simulink model "ATOM_simple_planning_simulator"  (R2026a)
settings: Solver=ode4  StopTime=100  FixedStep=0.01
StopFcn:
  | % Put every new figure in the same MATLAB Figures window as a docked tab.
  | set(groot, 'defaultFigureWindowStyle', 'docked');
  | 
  | if exist('costmap_active', 'var') && ...
  |     exist('vehicle', 'var') && ...
  |     exist('parking_path', 'var') && ...
  |     ~isempty(parking_path)
  | 
  |      plotPlan(costmap_active, vehicle, parking_path);
  | 
  |  else
  | 
  |      warning('No valid parking path is available for plotting.');
  | 
  |  end
  | 
  |  PlotControllerReferences( ...
  |      out.controller_reference_log);
  | 
  |  PlotControllerTracking( ...
  |      out.controller_tracking_log);
  | 
model workspace (MAT data in the model file):
  vehicle : object (value not decoded)
symbols that are objects in the model workspace (value not decoded): vehicle
undefined symbols (not defined in the file): delta_f_LUT, gain4WS_LUT, k_ref_LUT, kappa_gain_BP, Ki, Kp, lateral, longitudinal, planning_validator, rr_gain_BP, rr_LUT, stanley, velocity_smoother
libraries: slpidlib x1
(part 2 of 8)

== system ATOM_simple_planning_simulator/Lateral run()/SetStanleyTrajectory ==
  ref_traj : Inport
  ego_pose : Inport  Port=2
  Constant1 : Constant  Value=stanley.traj_resample_dist
  Resample Trajectory : MATLAB Function  TreatAsAtomicUnit=on
  calcLongOffsetToSegment : MATLAB Function  TreatAsAtomicUnit=on
  default : Constant  Value=3
  default1 : Constant  Value=pi/2
  findFirstNearestSegmentIndexWithSoftConstraints : MATLAB Function  TreatAsAtomicUnit=on
  trajectory_out : Outport
  wires:
  Constant1/1 -> Resample Trajectory/2(resample_interval_dist)
  calcLongOffsetToSegment/1(ego_offset_to_segment) -> Resample Trajectory/4(ego_offset_to_segment)
  ego_pose/1 -> findFirstNearestSegmentIndexWithSoftConstraints/4(pose), calcLongOffsetToSegment/2(ego_pose)
  findFirstNearestSegmentIndexWithSoftConstraints/1(nearest_seg_idx) -> calcLongOffsetToSegment/1(seg_idx), Resample Trajectory/3(nearest_seg_idx)
  default/1 -> findFirstNearestSegmentIndexWithSoftConstraints/2(dist_threshold)
  default1/1 -> findFirstNearestSegmentIndexWithSoftConstraints/3(yaw_threshold)
  Resample Trajectory/1(trajectory_out) -> trajectory_out/1
  ref_traj/1 -> Resample Trajectory/1(trajectory_in), calcLongOffsetToSegment/3(trajectory), findFirstNearestSegmentIndexWithSoftConstraints/1(trajectory)

== system ATOM_simple_planning_simulator/Parking Scenario2/Costmap generation: complex parking situation ==
  From Workspace1 : FromWorkspace  VariableName=veh
  MATLAB Function : MATLAB Function  TreatAsAtomicUnit=on
  costmap : Outport
  start_pose : Outport  Port=2
  goal_pose : Outport  Port=3
  wires:
  MATLAB Function/1(costmap) -> costmap/1
  From Workspace1/1 -> MATLAB Function/1(veh)
  MATLAB Function/2(start_pose) -> start_pose/1
  MATLAB Function/3(goal_pose) -> goal_pose/1

== system ATOM_simple_planning_simulator/Parking Scenario2/Costmap generation: corridor occupancy grid ==
  From Workspace1 : FromWorkspace  VariableName=veh
  MATLAB Function : MATLAB Function  TreatAsAtomicUnit=on
  costmap : Outport
  start_pose : Outport  Port=2
  goal_pose : Outport  Port=3
  wires:
  MATLAB Function/1(costmap) -> costmap/1
  From Workspace1/1 -> MATLAB Function/1(veh)
  MATLAB Function/3(goal_pose) -> goal_pose/1
  MATLAB Function/2(start_pose) -> start_pose/1

== system ATOM_simple_planning_simulator/Parking Scenario2/Costmap generation: empty occupancy grid ==
  From Workspace1 : FromWorkspace  VariableName=veh
  MATLAB Function : MATLAB Function  TreatAsAtomicUnit=on
  costmap : Outport
  start_pose : Outport  Port=2
  goal_pose : Outport  Port=3
  wires:
  MATLAB Function/1(costmap) -> costmap/1
  From Workspace1/1 -> MATLAB Function/1(veh)
  MATLAB Function/2(start_pose) -> start_pose/1
  MATLAB Function/3(goal_pose) -> goal_pose/1

== system ATOM_simple_planning_simulator/Parking Scenario2/Costmap generation: obstacle ==
  From Workspace1 : FromWorkspace  VariableName=veh
  MATLAB Function : MATLAB Function  TreatAsAtomicUnit=on
  costmap : Outport
  start_pose : Outport  Port=2
  goal_pose : Outport  Port=3
  wires:
  MATLAB Function/1(costmap) -> costmap/1
  From Workspace1/1 -> MATLAB Function/1(veh)
  MATLAB Function/2(start_pose) -> start_pose/1
  MATLAB Function/3(goal_pose) -> goal_pose/1

== system ATOM_simple_planning_simulator/Parking Scenario2/Costmap generation: obstacle1 ==
  From Workspace1 : FromWorkspace  VariableName=veh
  MATLAB Function : MATLAB Function  TreatAsAtomicUnit=on
  costmap : Outport
  start_pose : Outport  Port=2
  goal_pose : Outport  Port=3
  wires:
  MATLAB Function/1(costmap) -> costmap/1
  From Workspace1/1 -> MATLAB Function/1(veh)
  MATLAB Function/2(start_pose) -> start_pose/1
  MATLAB Function/3(goal_pose) -> goal_pose/1

== system ATOM_simple_planning_simulator/Parking Scenario2/Costmap generation: obstacle2 ==
  From Workspace1 : FromWorkspace  VariableName=veh
  MATLAB Function : MATLAB Function  TreatAsAtomicUnit=on
  costmap : Outport
  start_pose : Outport  Port=2
  goal_pose : Outport  Port=3
  wires:
  MATLAB Function/1(costmap) -> costmap/1
  From Workspace1/1 -> MATLAB Function/1(veh)
  MATLAB Function/2(start_pose) -> start_pose/1
  MATLAB Function/3(goal_pose) -> goal_pose/1

== system ATOM_simple_planning_simulator/Parking Scenario2/Costmap generation: parking scenario beside a lane ==
  From Workspace1 : FromWorkspace  VariableName=veh
  MATLAB Function : MATLAB Function  TreatAsAtomicUnit=on
  costmap : Outport
  start_pose : Outport  Port=2
  goal_pose : Outport  Port=3
  wires:
  MATLAB Function/1(costmap) -> costmap/1
  From Workspace1/1 -> MATLAB Function/1(veh)
  MATLAB Function/2(start_pose) -> start_pose/1
  MATLAB Function/3(goal_pose) -> goal_pose/1

== system ATOM_simple_planning_simulator/Parking Scenario2/Costmap generation: perpendicular lot ==
  From Workspace1 : FromWorkspace  VariableName=veh
  Perpendicular Parking : MATLAB Function  TreatAsAtomicUnit=on
  costmap : Outport
  start_pose : Outport  Port=2
  goal_pose : Outport  Port=3
  wires:
  Perpendicular Parking/1(costmap) -> costmap/1
  From Workspace1/1 -> Perpendicular Parking/1(veh)
  Perpendicular Parking/2(start_pose) -> start_pose/1
  Perpendicular Parking/3(goal_pose) -> goal_pose/1

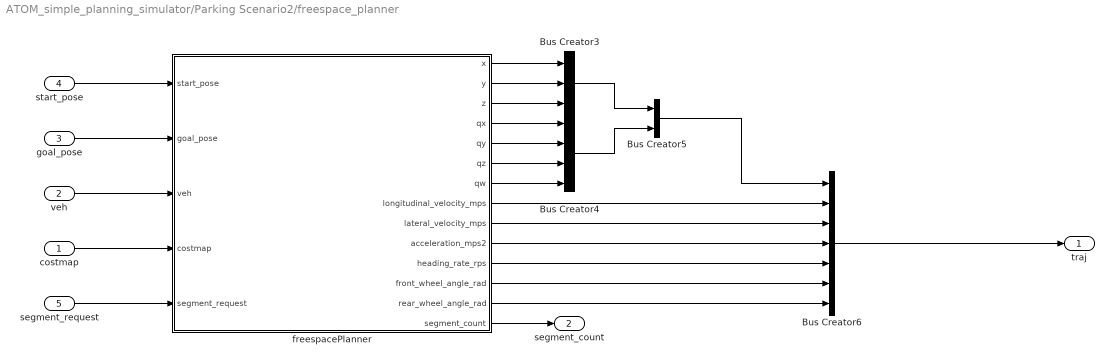
== system ATOM_simple_planning_simulator/Parking Scenario2/freespace_planner ==
  costmap : Inport
  veh : Inport  Port=2
  goal_pose : Inport  Port=3
  start_pose : Inport  Port=4
  segment_request : Inport  Port=5
  Bus Creator3 : BusCreator  Inputs=3  OutDataTypeStr=Bus: PointBusN
  Bus Creator4 : BusCreator  Inputs=4  OutDataTypeStr=Bus: QuaternionBusN
  Bus Creator5 : BusCreator  Inputs=2  OutDataTypeStr=Bus: PoseBusN
      settings: InheritFromInputs=off
  Bus Creator6 : BusCreator  Inputs=7  OutDataTypeStr=Bus: TrajectoryDataBus
      settings: InheritFromInputs=off
  freespacePlanner : MATLAB Function  TreatAsAtomicUnit=on
  traj : Outport
  segment_count : Outport  Port=2
  wires:
  Bus Creator6/1 -> traj/1
  Bus Creator3/1 -> Bus Creator5/1
  freespacePlanner/13(rear_wheel_angle_rad) -> Bus Creator6/7
  Bus Creator5/1 -> Bus Creator6/1
  freespacePlanner/8(longitudinal_velocity_mps) -> Bus Creator6/2
  freespacePlanner/3(z) -> Bus Creator3/3
  freespacePlanner/4(qx) -> Bus Creator4/1
  freespacePlanner/9(lateral_velocity_mps) -> Bus Creator6/3
  freespacePlanner/10(acceleration_mps2) -> Bus Creator6/4
  freespacePlanner/5(qy) -> Bus Creator4/2
  freespacePlanner/1(x) -> Bus Creator3/1
  freespacePlanner/2(y) -> Bus Creator3/2
  freespacePlanner/7(qw) -> Bus Creator4/4
  freespacePlanner/6(qz) -> Bus Creator4/3
  freespacePlanner/12(front_wheel_angle_rad) -> Bus Creator6/6
  Bus Creator4/1 -> Bus Creator5/2
  freespacePlanner/11(heading_rate_rps) -> Bus Creator6/5
  costmap/1 -> freespacePlanner/4(costmap)
  start_pose/1 -> freespacePlanner/1(start_pose)
  goal_pose/1 -> freespacePlanner/2(goal_pose)
  veh/1 -> freespacePlanner/3(veh)
  segment_request/1 -> freespacePlanner/5(segment_request)
  freespacePlanner/14(segment_count) -> segment_count/1

== system ATOM_simple_planning_simulator/Plot vehicle/SetStanleyTrajectory ==
  ref_traj : Inport
  ego_pose : Inport  Port=2
  Constant1 : Constant  Value=stanley.traj_resample_dist
  Resample Trajectory : MATLAB Function  TreatAsAtomicUnit=on
  calcLongOffsetToSegment : MATLAB Function  TreatAsAtomicUnit=on
  default : Constant  Value=3
  default1 : Constant  Value=pi/2
  findFirstNearestSegmentIndexWithSoftConstraints : MATLAB Function  TreatAsAtomicUnit=on
  trajectory_out : Outport
  wires:
  ref_traj/1 -> Resample Trajectory/1(trajectory_in), calcLongOffsetToSegment/3(trajectory), findFirstNearestSegmentIndexWithSoftConstraints/1(trajectory)
  Constant1/1 -> Resample Trajectory/2(resample_interval_dist)
  calcLongOffsetToSegment/1(ego_offset_to_segment) -> Resample Trajectory/4(ego_offset_to_segment)
  ego_pose/1 -> findFirstNearestSegmentIndexWithSoftConstraints/4(pose), calcLongOffsetToSegment/2(ego_pose)
  findFirstNearestSegmentIndexWithSoftConstraints/1(nearest_seg_idx) -> calcLongOffsetToSegment/1(seg_idx), Resample Trajectory/3(nearest_seg_idx)
  default/1 -> findFirstNearestSegmentIndexWithSoftConstraints/2(dist_threshold)
  default1/1 -> findFirstNearestSegmentIndexWithSoftConstraints/3(yaw_threshold)
  Resample Trajectory/1(trajectory_out) -> trajectory_out/1

== system ATOM_simple_planning_simulator/Plot vehicle3/SetStanleyTrajectory ==
  ref_traj : Inport
  ego_pose : Inport  Port=2
  Constant1 : Constant  Value=stanley.traj_resample_dist
  Resample Trajectory : MATLAB Function  TreatAsAtomicUnit=on
  calcLongOffsetToSegment : MATLAB Function  TreatAsAtomicUnit=on
  default : Constant  Value=3
  default1 : Constant  Value=pi/2
  findFirstNearestSegmentIndexWithSoftConstraints : MATLAB Function  TreatAsAtomicUnit=on
  trajectory_out : Outport
  wires:
  ref_traj/1 -> Resample Trajectory/1(trajectory_in), calcLongOffsetToSegment/3(trajectory), findFirstNearestSegmentIndexWithSoftConstraints/1(trajectory)
  Constant1/1 -> Resample Trajectory/2(resample_interval_dist)
  calcLongOffsetToSegment/1(ego_offset_to_segment) -> Resample Trajectory/4(ego_offset_to_segment)
  ego_pose/1 -> findFirstNearestSegmentIndexWithSoftConstraints/4(pose), calcLongOffsetToSegment/2(ego_pose)
  findFirstNearestSegmentIndexWithSoftConstraints/1(nearest_seg_idx) -> calcLongOffsetToSegment/1(seg_idx), Resample Trajectory/3(nearest_seg_idx)
  default/1 -> findFirstNearestSegmentIndexWithSoftConstraints/2(dist_threshold)
  default1/1 -> findFirstNearestSegmentIndexWithSoftConstraints/3(yaw_threshold)
  Resample Trajectory/1(trajectory_out) -> trajectory_out/1

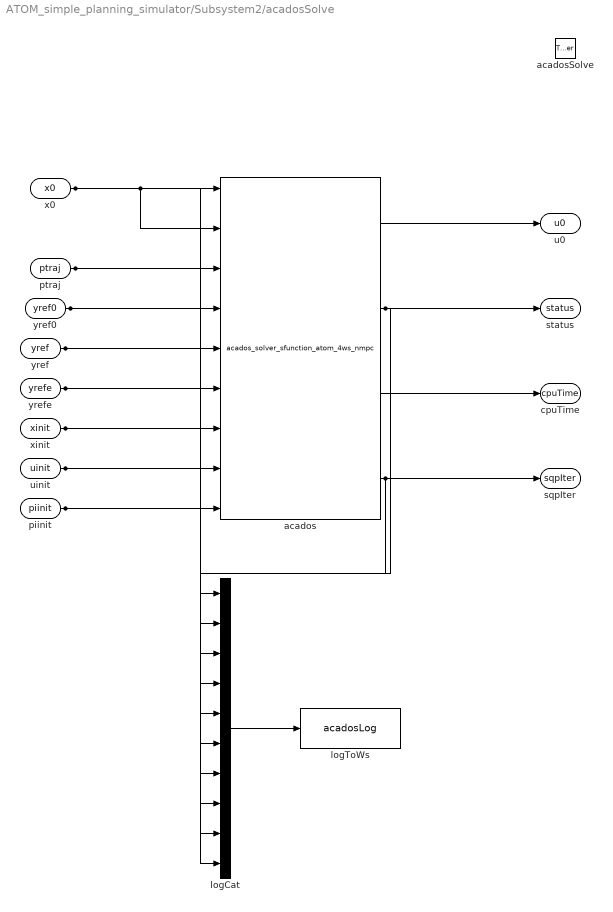
== system ATOM_simple_planning_simulator/Subsystem2/acadosSolve ==
  acadosSolve : TriggerPort  TriggerType=function-call  IsSimulinkFunction=on  FunctionName=acadosSolve  FunctionVisibility=scoped  VariantControl=(inherit)
  acados : S-Function  FunctionName=acados_solver_sfunction_atom_4ws_nmpc  SFunctionDeploymentMode=off  EnableBusSupport=off
  logCat : Concatenate  NumInputs=10
  logToWs : ToWorkspace  VariableName=acadosLog  SaveFormat=Structure With Time  SampleTime=-1
  x0 : ArgIn  DisableCoverage=on  PortDimensions=[9 1]  ArgumentName=x0
  ptraj : ArgIn  Port=2  PortDimensions=[272 1]  ArgumentName=ptraj
  yref0 : ArgIn  Port=3  PortDimensions=[7 1]  ArgumentName=yref0
  yref : ArgIn  Port=4  PortDimensions=[98 1]  ArgumentName=yref
  yrefe : ArgIn  Port=5  PortDimensions=[5 1]  ArgumentName=yrefe
  xinit : ArgIn  Port=6  PortDimensions=[144 1]  ArgumentName=xinit
  uinit : ArgIn  Port=7  PortDimensions=[30 1]  ArgumentName=uinit
  piinit : ArgIn  Port=8  PortDimensions=[135 1]  ArgumentName=piinit
  u0 : ArgOut  DisableCoverage=on  PortDimensions=[2 1]  ArgumentName=u0
  status : ArgOut  Port=2  ArgumentName=status
  cpuTime : ArgOut  Port=3  ArgumentName=cpuTime
  sqpIter : ArgOut  Port=4  ArgumentName=sqpIter
  wires:
  x0/1 -> acados/1, acados/2, logCat/1
  ptraj/1 -> acados/3, logCat/2
  yref0/1 -> acados/4, logCat/3
  yref/1 -> acados/5, logCat/4
  yrefe/1 -> acados/6, logCat/5
  xinit/1 -> acados/7, logCat/6
  uinit/1 -> acados/8, logCat/7
  piinit/1 -> acados/9, logCat/8
  acados/1 -> u0/1
  acados/2 -> status/1, logCat/9
  acados/3 -> cpuTime/1
  acados/4 -> sqpIter/1, logCat/10
  logCat/1 -> logToWs/1

== system ATOM_simple_planning_simulator/Vehicle Model/Vehicle Dynamics ==
  command : Inport
  rear_steer_command : Inport  Port=2
  From Workspace : FromWorkspace  VariableName=veh
  MATLAB Function : MATLAB Function  TreatAsAtomicUnit=on
  state integrator : Subsystem
  IntState : Outport
  wires:
  command/1 -> MATLAB Function/2(command)
  MATLAB Function/1(d_state) -> state integrator/1(d_state)  "d_state"
  state integrator/1(state) -> MATLAB Function/1(state), IntState/1
  From Workspace/1 -> MATLAB Function/3(veh)
  rear_steer_command/1 -> MATLAB Function/4(rear_steering_command)

== system ATOM_simple_planning_simulator/Vehicle Model/Vehicle internal state ==
  IntState : Inport
  Bus Selector : BusSelector  OutputSignals=x,y,yaw,vx,steer_front,steer_rear,acc
  Scope{,1..6} (7 alike) : Scope
      Scope settings: ActiveDisplayYMinimum=-1  ActiveDisplayYMaximum=1
      Scope1 settings: ActiveDisplayYMinimum=-1  ActiveDisplayYMaximum=1
      Scope2 settings: ActiveDisplayYMinimum=-1  ActiveDisplayYMaximum=1  DataLoggingVariableName=ScopeData2
      Scope3 settings: ActiveDisplayYMinimum=-1  ActiveDisplayYMaximum=1  DataLoggingVariableName=ScopeData3
      Scope4 settings: ActiveDisplayYMinimum=-1  ActiveDisplayYMaximum=1  DataLoggingVariableName=ScopeData4
      Scope5 settings: ActiveDisplayYMinimum=-1  ActiveDisplayYMaximum=1  DataLoggingVariableName=ScopeData5
      Scope6 settings: ActiveDisplayYMinimum=-1  ActiveDisplayYMaximum=1  DataLoggingVariableName=ScopeData6
  steer_front : Outport
  steer_rear : Outport  Port=2
  wires:
  Bus Selector/2 -> Scope1/1  "<y>"
  Bus Selector/4 -> Scope3/1  "<vx>"
  Bus Selector/1 -> Scope/1  "<x>"
  Bus Selector/3 -> Scope2/1  "<yaw>"
  Bus Selector/7 -> Scope6/1  "<acc>"
  Bus Selector/5 -> steer_front/1, Scope4/1  "<steer_front>"
  Bus Selector/6 -> steer_rear/1, Scope5/1  "<steer_rear>"
  IntState/1 -> Bus Selector/1

== system ATOM_simple_planning_simulator/Vehicle_Model2/Vehicle Dynamics ==
  command : Inport
  rear_steer_command : Inport  Port=2
  From Workspace : FromWorkspace  VariableName=veh
  MATLAB Function : MATLAB Function  TreatAsAtomicUnit=on
  state integrator : Subsystem
  IntState : Outport
  wires:
  command/1 -> MATLAB Function/2(command)
  MATLAB Function/1(d_state) -> state integrator/1(d_state)  "d_state"
  state integrator/1(state) -> MATLAB Function/1(state), IntState/1
  From Workspace/1 -> MATLAB Function/3(veh)
  rear_steer_command/1 -> MATLAB Function/4(rear_steering_command)

== system ATOM_simple_planning_simulator/Vehicle_Model2/Vehicle internal state ==
  IntState : Inport
  Bus Selector : BusSelector  OutputSignals=x,y,yaw,vx,steer_front,steer_rear,acc
  Scope{,1..6} (7 alike) : Scope
      Scope settings: ActiveDisplayYMinimum=-1  ActiveDisplayYMaximum=1
      Scope1 settings: ActiveDisplayYMinimum=-1  ActiveDisplayYMaximum=1
      Scope2 settings: ActiveDisplayYMinimum=-1  ActiveDisplayYMaximum=1  DataLoggingVariableName=ScopeData2
      Scope3 settings: ActiveDisplayYMinimum=-1  ActiveDisplayYMaximum=1  DataLoggingVariableName=ScopeData3
      Scope4 settings: ActiveDisplayYMinimum=-1  ActiveDisplayYMaximum=1  DataLoggingVariableName=ScopeData4
      Scope5 settings: ActiveDisplayYMinimum=-1  ActiveDisplayYMaximum=1  DataLoggingVariableName=ScopeData5
      Scope6 settings: ActiveDisplayYMinimum=-1  ActiveDisplayYMaximum=1  DataLoggingVariableName=ScopeData6
  steer_front : Outport
  steer_rear : Outport  Port=2
  wires:
  Bus Selector/2 -> Scope1/1  "<y>"
  Bus Selector/4 -> Scope3/1  "<vx>"
  Bus Selector/1 -> Scope/1  "<x>"
  Bus Selector/3 -> Scope2/1  "<yaw>"
  Bus Selector/7 -> Scope6/1  "<acc>"
  Bus Selector/5 -> steer_front/1, Scope4/1  "<steer_front>"
  Bus Selector/6 -> steer_rear/1, Scope5/1  "<steer_rear>"
  IntState/1 -> Bus Selector/1

== system ATOM_simple_planning_simulator/trajectory_checker plugin - planning_validator_node/check_valid_steering ==
  trajectory : Inport
  veh : Inport  Port=2
  CheckValidSteering : MATLAB Function  TreatAsAtomicUnit=on
  Constant : Constant  Value=planning_validator.steering.threshold
  calcMaxSteeringAngles : Subsystem
  is_valid_steering : Outport
  wires:
  calcMaxSteeringAngles/1(max_steering) -> CheckValidSteering/1(max_steering)
  calcMaxSteeringAngles/2(i) -> ?
  Constant/1 -> CheckValidSteering/2(steering_threshold)
  CheckValidSteering/1(is_valid_steering) -> is_valid_steering/1
  trajectory/1 -> calcMaxSteeringAngles/1(trajectory)
  veh/1 -> calcMaxSteeringAngles/2(veh)

== system ATOM_simple_planning_simulator/trajectory_checker plugin - planning_validator_node/check_valid_steering_rate ==
  trajectory : Inport
  veh : Inport  Port=2
  CheckValidSteeringRate : MATLAB Function  TreatAsAtomicUnit=on
  Constant : Constant  Value=planning_validator.steering_rate.threshold
  calcMaxSteeringRates : Subsystem
  is_valid_steering_rate : Outport
  wires:
  calcMaxSteeringRates/1(max_steering_rate) -> CheckValidSteeringRate/1(max_steering_rate)
  calcMaxSteeringRates/2(i) -> ?
  Constant/1 -> CheckValidSteeringRate/2(steering_rate_threshold)
  CheckValidSteeringRate/1(is_valid_steering_rate) -> is_valid_steering_rate/1
  trajectory/1 -> calcMaxSteeringRates/1(trajectory)
  veh/1 -> calcMaxSteeringRates/2(veh)

== system ATOM_simple_planning_simulator/velocity_smoother_node/ApplyLateralAccelerationFilter - velocity_smoother node ==
  curvature : Inport
  "trajectory " : Inport  Port=2
  ComputeVelocityProfile and Acceleration : MATLAB Function  TreatAsAtomicUnit=on
  Constant : Constant  Value=velocity_smoother.lateral_acceleration_limits(1)
  Constant1 : Constant  Value=velocity_smoother.min_curve_velocity
  Constant2 : Constant  Value=0.5
  MATLAB Function1 : MATLAB Function  TreatAsAtomicUnit=on
  abs(velocity_smoother.min_acc) : Constant  Value=abs(velocity_smoother.min_acc)
  velocity_smoother.max_acc : Constant  Value=velocity_smoother.max_acc
  velocity_smoother.v_end : Constant  Value=velocity_smoother.v_end
  velocity_smoother.v_start : Constant  Value=velocity_smoother.v_start
  trajectory : Outport
  wires:
  velocity_smoother.v_end/1 -> ComputeVelocityProfile and Acceleration/4(v_end)
  ComputeVelocityProfile and Acceleration/1(trajectory) -> trajectory/1
  curvature/1 -> MATLAB Function1/3(curvature)
  velocity_smoother.v_start/1 -> ComputeVelocityProfile and Acceleration/3(v_start)
  velocity_smoother.max_acc/1 -> ComputeVelocityProfile and Acceleration/1(a_accel_max)
  abs(velocity_smoother.min_acc)/1 -> ComputeVelocityProfile and Acceleration/2(a_decel_max)
  MATLAB Function1/1(trajectory) -> ComputeVelocityProfile and Acceleration/5("trajectory ")
  Constant2/1 -> MATLAB Function1/2(min_curve_velocity)
  Constant/1 -> MATLAB Function1/1(a_lat_max)
  "trajectory "/1 -> MATLAB Function1/4("trajectory ")

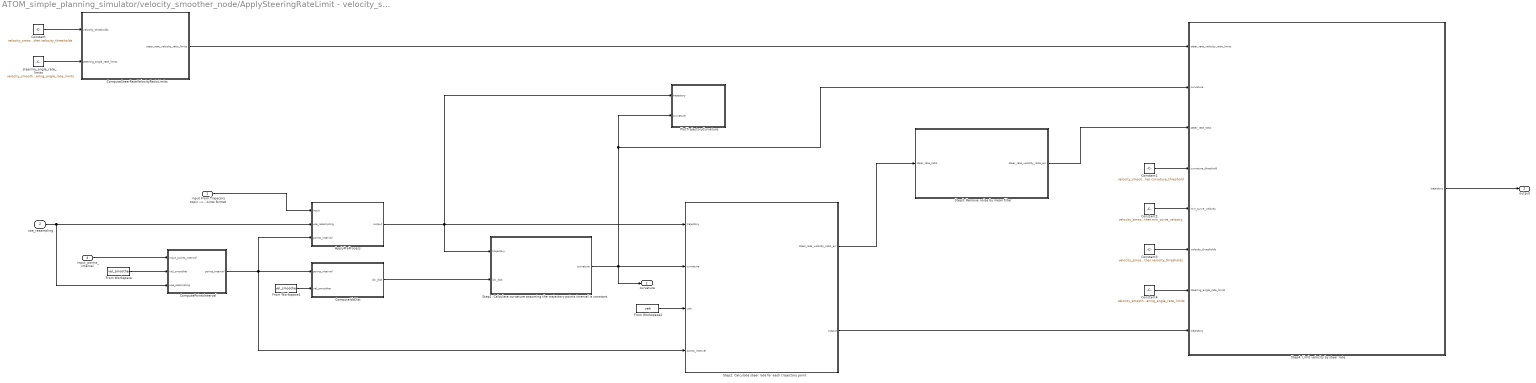
== system ATOM_simple_planning_simulator/velocity_smoother_node/ApplySteeringRateLimit - velocity_smoother_node ==
  input From Trajecory topic --> TrajectoryPoints format : Inport
  use_resampling : Inport  Port=2
  input_points_interval : Inport  Port=3
  ApplyPreProcess : MATLAB Function  TreatAsAtomicUnit=on
  ComputeIdxDist : MATLAB Function  TreatAsAtomicUnit=on
  ComputePointsInterval : MATLAB Function  TreatAsAtomicUnit=on
  ComputeSteerRateVelocityRatioLimits : MATLAB Function  TreatAsAtomicUnit=on
  Constant : Constant  Value=velocity_smoother.velocity_thresholds
  Constant1 : Constant  Value=velocity_smoother.curvature_threshold
  Constant2 : Constant  Value=velocity_smoother.min_curve_velocity
  Constant3 : Constant  Value=velocity_smoother.velocity_thresholds
  Constant4 : Constant  Value=velocity_smoother.steering_angle_rate_limits
  From Workspace : FromWorkspace  VariableName=vel_smoother
  From Workspace1 : FromWorkspace  VariableName=vel_smoother
  From Workspace2 : FromWorkspace  VariableName=veh
  PlotTrajectoryCurvature : MATLAB Function  TreatAsAtomicUnit=on
  Step1: Calculate curvature assuming the trajectory points interval is constant. : Subsystem
  Step2: Calculate steer rate for each trajectory point : Subsystem
  Step3: Remove noise by mean filter : Subsystem
  Step4: Limit velocity by steer rate. : Subsystem
  steering_angle_rate_limits : Constant  Value=velocity_smoother.steering_angle_rate_limits
  curvature : Outport
  output : Outport  Port=2
  wires:
  use_resampling/1 -> ApplyPreProcess/2(use_resempling), ComputePointsInterval/3(use_resampling)
  input From Trajecory topic --> TrajectoryPoints format/1 -> ApplyPreProcess/1(input)
  input_points_interval/1 -> ComputePointsInterval/1(input_points_interval)
  ComputePointsInterval/1(points_interval) -> Step2: Calculate steer rate for each trajectory point/4(points_interval), ComputeIdxDist/1(points_interval), ApplyPreProcess/3(points_interval)
  From Workspace/1 -> ComputePointsInterval/2(vel_smoother)
  From Workspace1/1 -> ComputeIdxDist/2(vel_smoother)
  ApplyPreProcess/1(output) -> PlotTrajectoryCurvature/1(trajectory), Step1: Calculate curvature assuming the trajectory points interval is constant./1(trajectory), Step2: Calculate steer rate for each trajectory point/1(trajectory)
  Step1: Calculate curvature assuming the trajectory points interval is constant./1(curvature) -> curvature/1, PlotTrajectoryCurvature/2(curvature), Step4: Limit velocity by steer rate./2(curvature), Step2: Calculate steer rate for each trajectory point/2(curvature)
  ComputeIdxDist/1(idx_dist) -> Step1: Calculate curvature assuming the trajectory points interval is constant./2(idx_dist)
  From Workspace2/1 -> Step2: Calculate steer rate for each trajectory point/3(veh)
  Step2: Calculate steer rate for each trajectory point/1(steer_rate_velocity_ratio_arr) -> Step3: Remove noise by mean filter/1(steer_rate_ratio)
  steering_angle_rate_limits/1 -> ComputeSteerRateVelocityRatioLimits/2(steering_angle_rate_limits)
  Constant/1 -> ComputeSteerRateVelocityRatioLimits/1(velocity_thresholds)
  ComputeSteerRateVelocityRatioLimits/1(steer_rate_velocity_ratio_limits) -> Step4: Limit velocity by steer rate./1(steer_rate_velocity_ratio_limits)
  Step3: Remove noise by mean filter/1(steer_rate_velocity_ratio_arr) -> Step4: Limit velocity by steer rate./3(steer_rate_ratio)
  Constant1/1 -> Step4: Limit velocity by steer rate./4(curvature_threshold)
  Constant2/1 -> Step4: Limit velocity by steer rate./5(min_curve_velocity)
  Constant3/1 -> Step4: Limit velocity by steer rate./6(velocity_thresholds)
  Constant4/1 -> Step4: Limit velocity by steer rate./7(steering_angle_rate_limits)
  Step2: Calculate steer rate for each trajectory point/2(output) -> Step4: Limit velocity by steer rate./8("trajectory ")
  Step4: Limit velocity by steer rate./1(trajectory) -> output/1

== system ATOM_simple_planning_simulator/Lateral run()/CalculateStanley/Stanley controller ==
  stanley_data : Inport
  Abs : Abs  SaturateOnIntegerOverflow=off
  Bus Selector : BusSelector  OutputSignals=ref_curvature
  Constant : Constant  Value=stanley.k_gain
  Constant1 : Constant  Value=stanley.k_soft
  Constant3 : Constant  Value=vehicle.param.max_steer_angle
  Constant4 : Constant  Value=vehicle.param.wheel_base
  calculateSteer - Stanley : MATLAB Function  TreatAsAtomicUnit=on
  gain_4WS = f(rr,k_ref) : Lookup_n-D  BreakpointsForDimension1=rr_gain_BP  BreakpointsForDimension2=kappa_gain_BP  Table=gain4WS_LUT  InternalRulePriority=Speed  RndMeth=Simplest
      settings: InputPortMap=u0,u1
  rr = f(k_ref) : Lookup_n-D  NumberOfTableDimensions=1  BreakpointsForDimension1=k_ref_LUT  Table=rr_LUT  InternalRulePriority=Speed  RndMeth=Simplest
  steering_cmd : Outport
  rear_steer : Outport  Port=2
  wires:
  Constant1/1 -> calculateSteer - Stanley/5(k_soft)
  Constant/1 -> calculateSteer - Stanley/4(k_gain)
  stanley_data/1 -> calculateSteer - Stanley/1(stanley_data), Bus Selector/1
  calculateSteer - Stanley/1(front_steer) -> steering_cmd/1
  Constant4/1 -> calculateSteer - Stanley/2(wheelbase)
  gain_4WS = f(rr,k_ref)/1 -> calculateSteer - Stanley/7(gain_4WS)
  calculateSteer - Stanley/2(rear_steer) -> rear_steer/1
  Bus Selector/1 -> Abs/1  "<ref_curvature>"
  rr = f(k_ref)/1 -> gain_4WS = f(rr,k_ref)/1, calculateSteer - Stanley/6(rr)
  Constant3/1 -> calculateSteer - Stanley/3(steer_limit)
  Abs/1 -> gain_4WS = f(rr,k_ref)/2, rr = f(k_ref)/1

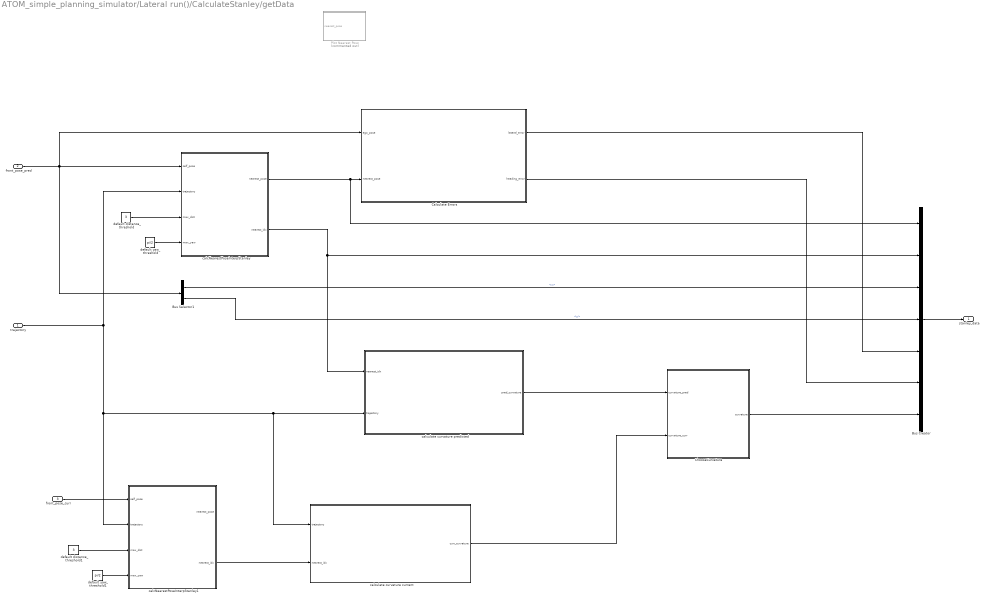
== system ATOM_simple_planning_simulator/Lateral run()/CalculateStanley/getData ==
  trajectory : Inport
  front_pose_pred : Inport  Port=2
  front_pose_curr : Inport  Port=3
  Bus Creator : BusCreator  Inputs=7  OutDataTypeStr=Bus: StanleyInputDataBus
      settings: InheritFromInputs=off
  Bus Selector1 : BusSelector  OutputSignals=twist.linear.x,twist.linear.y
  Calculate Errors : Subsystem
  ChooseCurvature : MATLAB Function  TreatAsAtomicUnit=on
  Plot Nearest Pose : MATLAB Function  Commented=on  TreatAsAtomicUnit=on
  calcNearestPoseInterpStanley : MATLAB Function  TreatAsAtomicUnit=on
  calcNearestPoseInterpStanley1 : MATLAB Function  TreatAsAtomicUnit=on
  calculate curvature current : Subsystem
  calculate curvature predicted : Subsystem
  default distance_threshold : Constant  Value=3
  default distance_threshold1 : Constant  Value=3
  default yaw_threshold : Constant  Value=pi/2
  default yaw_threshold1 : Constant  Value=pi/2
  stanley_data : Outport
  wires:
  default distance_threshold/1 -> calcNearestPoseInterpStanley/3(max_dist)
  default yaw_threshold/1 -> calcNearestPoseInterpStanley/4(max_yaw)
  front_pose_pred/1 -> Bus Selector1/1, Calculate Errors/1(ego_pose), calcNearestPoseInterpStanley/1(self_pose)
  calcNearestPoseInterpStanley/2(nearest_idx) -> calculate curvature predicted/1(nearest_idx), Bus Creator/2
  Bus Creator/1 -> stanley_data/1
  Bus Selector1/1 -> Bus Creator/3  "<x>"
  Calculate Errors/1(lateral_error) -> Bus Creator/5
  Calculate Errors/2(heading_error) -> Bus Creator/6
  calculate curvature predicted/1(pred_curvature) -> ChooseCurvature/1(curvature_pred)
  front_pose_curr/1 -> calcNearestPoseInterpStanley1/1(self_pose)
  default distance_threshold1/1 -> calcNearestPoseInterpStanley1/3(max_dist)
  default yaw_threshold1/1 -> calcNearestPoseInterpStanley1/4(max_yaw)
  calcNearestPoseInterpStanley1/2(nearest_idx) -> calculate curvature current/2(nearest_idx)
  trajectory/1 -> calcNearestPoseInterpStanley/2(trajectory), calcNearestPoseInterpStanley1/2(trajectory), calculate curvature current/1(trajectory), calculate curvature predicted/2(trajectory)
  calculate curvature current/1(curr_curvature) -> ChooseCurvature/2(curvature_curr)
  ChooseCurvature/1(curvature) -> Bus Creator/7
  calcNearestPoseInterpStanley/1(nearest_pose) -> Bus Creator/1, Calculate Errors/2(nearest_pose)
  Bus Selector1/2 -> Bus Creator/4  "<y>"

== system ATOM_simple_planning_simulator/Vehicle Model/Vehicle Dynamics/state integrator ==
  d_state : Inport
  Bus Creator : BusCreator  Inputs=7  OutDataTypeStr=Bus: VehicleInternalStateBus
      settings: InheritFromInputs=off
  Bus Selector : BusSelector  OutputSignals=acc,steer_rear,steer_front,vx,yaw,y,x
  Integrator{,1..5} (6 alike) : Integrator
  Integrator6 : Integrator  InitialCondition=-2
  state : Outport
  wires:
  Integrator4/1 -> Bus Creator/3
  Integrator3/1 -> Bus Creator/4
  Integrator6/1 -> Bus Creator/1
  Bus Selector/4 -> Integrator3/1  "<vx>"
  Integrator1/1 -> Bus Creator/6
  Bus Creator/1 -> state/1
  Bus Selector/6 -> Integrator5/1  "<y>"
  Bus Selector/2 -> Integrator1/1  "<steer_rear>"
  Integrator5/1 -> Bus Creator/2
  Bus Selector/7 -> Integrator6/1  "<x>"
  Bus Selector/3 -> Integrator2/1  "<steer_front>"
  Bus Selector/1 -> Integrator/1  "<acc>"
  Integrator/1 -> Bus Creator/7
  Bus Selector/5 -> Integrator4/1  "<yaw>"
  d_state/1 -> Bus Selector/1
  Integrator2/1 -> Bus Creator/5

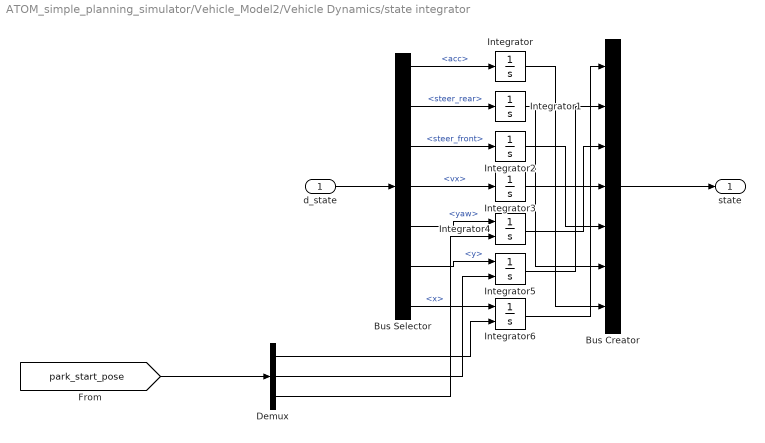
== system ATOM_simple_planning_simulator/Vehicle_Model2/Vehicle Dynamics/state integrator ==
  d_state : Inport
  Bus Creator : BusCreator  Inputs=7  OutDataTypeStr=Bus: VehicleInternalStateBus
      settings: InheritFromInputs=off
  Bus Selector : BusSelector  OutputSignals=acc,steer_rear,steer_front,vx,yaw,y,x
  Demux : Demux  Outputs=3
  Integrator{,1..3} (4 alike) : Integrator
  Integrator4 : Integrator  InitialConditionSource=external
  Integrator5 : Integrator  InitialConditionSource=external
  Integrator6 : Integrator  InitialConditionSource=external  InitialCondition=-2
  state : Outport
  wires:
  Integrator4/1 -> Bus Creator/3
  Integrator3/1 -> Bus Creator/4
  Integrator6/1 -> Bus Creator/1
  Bus Selector/4 -> Integrator3/1  "<vx>"
  Integrator1/1 -> Bus Creator/6
  Bus Creator/1 -> state/1
  Bus Selector/6 -> Integrator5/1  "<y>"
  Bus Selector/2 -> Integrator1/1  "<steer_rear>"
  Integrator5/1 -> Bus Creator/2
  Bus Selector/7 -> Integrator6/1  "<x>"
  Bus Selector/3 -> Integrator2/1  "<steer_front>"
  Bus Selector/1 -> Integrator/1  "<acc>"
  Integrator/1 -> Bus Creator/7
  Bus Selector/5 -> Integrator4/1  "<yaw>"
  d_state/1 -> Bus Selector/1
  Integrator2/1 -> Bus Creator/5
  [park_start_pose] -> Demux/1
  Demux/1 -> Integrator6/2
  Demux/2 -> Integrator5/2
  Demux/3 -> Integrator4/2

== system ATOM_simple_planning_simulator/trajectory_checker plugin - planning_validator_node/check_valid_steering/calcMaxSteeringAngles ==
  trajectory : Inport
  veh : Inport  Port=2
  DecideValIdx : MATLAB Function  TreatAsAtomicUnit=on
  GetAbsMaxValAndIdx front : MATLAB Function  TreatAsAtomicUnit=on
  GetAbsMaxValAndIdx rear : MATLAB Function  TreatAsAtomicUnit=on
  calcSteeringAngles : Subsystem
  max_steering : Outport
  i : Outport  Port=2
  wires:
  trajectory/1 -> calcSteeringAngles/1(trajectory)
  veh/1 -> calcSteeringAngles/2(veh)
  calcSteeringAngles/2(rear_steering_vector) -> GetAbsMaxValAndIdx rear/1(values)
  calcSteeringAngles/1(front_steering_vector) -> GetAbsMaxValAndIdx front/1(values)
  GetAbsMaxValAndIdx front/1(max_value) -> DecideValIdx/1(max_front)
  GetAbsMaxValAndIdx rear/2(max_index) -> DecideValIdx/4(idx_rear)
  GetAbsMaxValAndIdx rear/1(max_value) -> DecideValIdx/3(max_rear)
  GetAbsMaxValAndIdx front/2(max_index) -> DecideValIdx/2(idx_front)
  DecideValIdx/1(max_steering) -> max_steering/1
  DecideValIdx/2(max_index) -> i/1

== system ATOM_simple_planning_simulator/trajectory_checker plugin - planning_validator_node/check_valid_steering_rate/calcMaxSteeringRates ==
  trajectory : Inport
  veh : Inport  Port=2
  DecideValIdx : MATLAB Function  TreatAsAtomicUnit=on
  MATLAB Function : MATLAB Function  TreatAsAtomicUnit=on
  MATLAB Function1 : MATLAB Function  TreatAsAtomicUnit=on
  calcSteeringAngles : Subsystem
  max_steering_rate : Outport
  i : Outport  Port=2
  wires:
  trajectory/1 -> MATLAB Function1/1(trajectory), MATLAB Function/1(trajectory), calcSteeringAngles/1(trajectory)
  veh/1 -> calcSteeringAngles/2(veh)
  DecideValIdx/1(max_steering_rate) -> max_steering_rate/1
  DecideValIdx/2(max_index) -> i/1
  calcSteeringAngles/1(front_steering_vector) -> MATLAB Function/2(steering_vector)
  calcSteeringAngles/2(rear_steering_vector) -> MATLAB Function1/2(steering_vector)
  MATLAB Function/1(max_steering_rate) -> DecideValIdx/1(max_front)
  MATLAB Function/2(max_index) -> DecideValIdx/2(idx_front)
  MATLAB Function1/1(max_steering_rate) -> DecideValIdx/3(max_rear)
  MATLAB Function1/2(max_index) -> DecideValIdx/4(idx_rear)

== system ATOM_simple_planning_simulator/velocity_smoother_node/ApplySteeringRateLimit - velocity_smoother_node/Step1: Calculate curvature assuming the trajectory points interval is constant. ==
  trajectory : Inport
  idx_dist : Inport  Port=2
  CalcTrajectoryCurvature : MATLAB Function  TreatAsAtomicUnit=on
  curvature : Outport
  wires:
  idx_dist/1 -> CalcTrajectoryCurvature/2(idx_dist)
  CalcTrajectoryCurvature/1(curvature) -> curvature/1
  trajectory/1 -> CalcTrajectoryCurvature/1(trajectory)

== system ATOM_simple_planning_simulator/velocity_smoother_node/ApplySteeringRateLimit - velocity_smoother_node/Step2: Calculate steer rate for each trajectory point ==
  trajectory : Inport
  curvature : Inport  Port=2
  veh : Inport  Port=3
  points_interval : Inport  Port=4
  ComputeSteeringRate4WS : MATLAB Function  TreatAsAtomicUnit=on
  Constant : Constant  Value=k_ref_LUT
  Constant1 : Constant  Value=rr_LUT
  Constant2 : Constant  Value=delta_f_LUT
  steer_rate_velocity_ratio_arr : Outport
  output : Outport  Port=2
  wires:
  curvature/1 -> ComputeSteeringRate4WS/2(curvature)
  trajectory/1 -> ComputeSteeringRate4WS/1(trajectory)
  points_interval/1 -> ComputeSteeringRate4WS/4(points_interval)
  veh/1 -> ComputeSteeringRate4WS/3(veh)
  ComputeSteeringRate4WS/1(steer_rate_velocity_ratio_arr) -> steer_rate_velocity_ratio_arr/1
  ComputeSteeringRate4WS/2(output) -> output/1
  Constant/1 -> ComputeSteeringRate4WS/5(k_ref_LUT)
  Constant1/1 -> ComputeSteeringRate4WS/6(rr_LUT)
  Constant2/1 -> ComputeSteeringRate4WS/7(delta_f_LUT)

== system ATOM_simple_planning_simulator/velocity_smoother_node/ApplySteeringRateLimit - velocity_smoother_node/Step3: Remove noise by mean filter ==
  steer_rate_ratio : Inport
  MeanFilterSteeringRateRato : MATLAB Function  TreatAsAtomicUnit=on
  steer_rate_velocity_ratio_arr : Outport
  wires:
  steer_rate_ratio/1 -> MeanFilterSteeringRateRato/1(steer_rate_ratio)
  MeanFilterSteeringRateRato/1(steer_rate_velocity_ratio_arr) -> steer_rate_velocity_ratio_arr/1

== system ATOM_simple_planning_simulator/velocity_smoother_node/ApplySteeringRateLimit - velocity_smoother_node/Step4: Limit velocity by steer rate. ==
  steer_rate_velocity_ratio_limits : Inport
  curvature : Inport  Port=2
  steer_rate_ratio : Inport  Port=3
  curvature_threshold : Inport  Port=4
  min_curve_velocity : Inport  Port=5
  velocity_thresholds : Inport  Port=6
  steering_angle_rate_limits : Inport  Port=7
  "trajectory " : Inport  Port=8
  ApplySteeringRateVelocityLimit : MATLAB Function  TreatAsAtomicUnit=on
  trajectory : Outport
  wires:
  velocity_thresholds/1 -> ApplySteeringRateVelocityLimit/6(velocity_thresholds)
  ApplySteeringRateVelocityLimit/1(trajectory) -> trajectory/1
  "trajectory "/1 -> ApplySteeringRateVelocityLimit/8("trajectory ")
  steer_rate_velocity_ratio_limits/1 -> ApplySteeringRateVelocityLimit/1(steer_rate_velocity_ratio_limits)
  curvature/1 -> ApplySteeringRateVelocityLimit/2(curvature)
  steer_rate_ratio/1 -> ApplySteeringRateVelocityLimit/3(steer_rate_ratio)
  steering_angle_rate_limits/1 -> ApplySteeringRateVelocityLimit/7(steering_angle_rate_limits)
  curvature_threshold/1 -> ApplySteeringRateVelocityLimit/4(curvature_threshold)
  min_curve_velocity/1 -> ApplySteeringRateVelocityLimit/5(min_curve_velocity)

== system ATOM_simple_planning_simulator/Lateral run()/CalculateStanley/getData/Calculate Errors ==
  ego_pose : Inport
  nearest_pose : Inport  Port=2
  Plot Stanley Errors : MATLAB Function  TreatAsAtomicUnit=on
  calcLateralErrorStanley : MATLAB Function  TreatAsAtomicUnit=on
  calcYawErrorStanley : MATLAB Function  TreatAsAtomicUnit=on
  lateral_error : Outport
  heading_error : Outport  Port=2
  wires:
  nearest_pose/1 -> calcYawErrorStanley/2(nearest_pose), calcLateralErrorStanley/2(nearest_pose)
  ego_pose/1 -> calcLateralErrorStanley/1(ego_pose), calcYawErrorStanley/1(ego_pose)
  calcYawErrorStanley/1(yaw_err) -> heading_error/1, Plot Stanley Errors/2(heading_error)
  calcLateralErrorStanley/1(lateral_error) -> lateral_error/1, Plot Stanley Errors/1(lateral_error)

== system ATOM_simple_planning_simulator/Lateral run()/CalculateStanley/getData/calculate curvature current ==
  trajectory : Inport
  nearest_idx : Inport  Port=2
  CalcTrajectoryCurvature : MATLAB Function  TreatAsAtomicUnit=on
  ComputeIdxDist : MATLAB Function  TreatAsAtomicUnit=on
  ComputePointsInterval : MATLAB Function  TreatAsAtomicUnit=on
  From Workspace : FromWorkspace  VariableName=vel_smoother
  From Workspace1 : FromWorkspace  VariableName=vel_smoother
  input_points_interval [m] : Constant  OutDataTypeStr=double
  use_resampling == false : Constant  Value=0  OutDataTypeStr=boolean
  curr_curvature : Outport
  wires:
  From Workspace1/1 -> ComputeIdxDist/2(vel_smoother)
  CalcTrajectoryCurvature/1(curvature) -> curr_curvature/1
  use_resampling == false/1 -> ComputePointsInterval/3(use_resampling)
  ComputePointsInterval/1(points_interval) -> ComputeIdxDist/1(points_interval)
  From Workspace/1 -> ComputePointsInterval/2(vel_smoother)
  input_points_interval [m]/1 -> ComputePointsInterval/1(input_points_interval)
  trajectory/1 -> CalcTrajectoryCurvature/1(trajectory)
  ComputeIdxDist/1(idx_dist) -> CalcTrajectoryCurvature/3(idx_dist)
  nearest_idx/1 -> CalcTrajectoryCurvature/2(nearest_idx)

== system ATOM_simple_planning_simulator/Lateral run()/CalculateStanley/getData/calculate curvature predicted ==
  nearest_idx : Inport
  trajectory : Inport  Port=2
  CalcTrajectoryCurvature : MATLAB Function  TreatAsAtomicUnit=on
  ComputeIdxDist : MATLAB Function  TreatAsAtomicUnit=on
  ComputePointsInterval : MATLAB Function  TreatAsAtomicUnit=on
  From Workspace : FromWorkspace  VariableName=vel_smoother
  From Workspace1 : FromWorkspace  VariableName=vel_smoother
  input_points_interval [m] : Constant  OutDataTypeStr=double
  use_resampling == false : Constant  Value=0  OutDataTypeStr=boolean
  pred_curvature : Outport
  wires:
  From Workspace1/1 -> ComputeIdxDist/2(vel_smoother)
  CalcTrajectoryCurvature/1(curvature) -> pred_curvature/1
  use_resampling == false/1 -> ComputePointsInterval/3(use_resampling)
  ComputePointsInterval/1(points_interval) -> ComputeIdxDist/1(points_interval)
  From Workspace/1 -> ComputePointsInterval/2(vel_smoother)
  input_points_interval [m]/1 -> ComputePointsInterval/1(input_points_interval)
  trajectory/1 -> CalcTrajectoryCurvature/1(trajectory)
  ComputeIdxDist/1(idx_dist) -> CalcTrajectoryCurvature/3(idx_dist)
  nearest_idx/1 -> CalcTrajectoryCurvature/2(nearest_idx)

== system ATOM_simple_planning_simulator/trajectory_checker plugin - planning_validator_node/check_valid_steering/calcMaxSteeringAngles/calcSteeringAngles ==
  trajectory : Inport
  veh : Inport  Port=2
  calcCurvature : MATLAB Function  TreatAsAtomicUnit=on
  steering_vector calculation : MATLAB Function  TreatAsAtomicUnit=on
  front_steering_vector : Outport
  rear_steering_vector : Outport  Port=2
  wires:
  steering_vector calculation/2(rear_steering_vector) -> rear_steering_vector/1
  veh/1 -> steering_vector calculation/2(veh)
  trajectory/1 -> calcCurvature/1(trajectory)
  calcCurvature/1(curvature_vector) -> steering_vector calculation/1(curvature)
  steering_vector calculation/1(front_steering_vector) -> front_steering_vector/1

== system ATOM_simple_planning_simulator/trajectory_checker plugin - planning_validator_node/check_valid_steering_rate/calcMaxSteeringRates/calcSteeringAngles ==
  trajectory : Inport
  veh : Inport  Port=2
  calcCurvature : MATLAB Function  TreatAsAtomicUnit=on
  steering_vector calculation : MATLAB Function  TreatAsAtomicUnit=on
  front_steering_vector : Outport
  rear_steering_vector : Outport  Port=2
  wires:
  steering_vector calculation/2(rear_steering_vector) -> rear_steering_vector/1
  veh/1 -> steering_vector calculation/2(veh)
  trajectory/1 -> calcCurvature/1(trajectory)
  calcCurvature/1(curvature_vector) -> steering_vector calculation/1(curvature)
  steering_vector calculation/1(front_steering_vector) -> front_steering_vector/1

== matlab function ATOM_simple_planning_simulator/Vehicle_Model2/localization//kinematic_state function ==
  data: state input Bus: VehicleInternalStateBus; kinematic output Bus: KinematicStateBus; veh input
function kinematic = IntStateToKinematicState(state, veh)


%% Vehicle parameters

L = veh(3);


%% Current state

x = state.x;
y = state.y;
yaw = state.yaw;



% NOTE:
% vx is the longitudinal velocity expressed in the vehicle body frame
% (base_link located at the center of the rear axle).
% The vehicle speed magnitude is reconstructed as
%
%   v = vx / cos(delta_r)
%
% under the pure-rolling assumption (alpha_f = alpha_r = 0).

vx = state.vx;

steer_front = state.steer_front;
steer_rear  = state.steer_rear;


%% Pose

kinematic.pose.position.x = x;
kinematic.pose.position.y = y;
kinematic.pose.position.z = 0;


[qx,qy,qz,qw] = yawToQuaternion(yaw);

% quaternion from yaw only

kinematic.pose.orientation.x = qx;
kinematic.pose.orientation.y = qy;
kinematic.pose.orientation.z = qz;
kinematic.pose.orientation.w = qw;



%% Twist

% Body frame velocity

kinematic.twist.linear.x = vx;

kinematic.twist.linear.y = ...              % Modified for 4WS considering beta = steer_rear
    vx*tan(steer_rear);

kinematic.twist.linear.z = 0;



% Angular velocity

kinematic.twist.angular.x = 0;
kinematic.twist.angular.y = 0;

kinematic.twist.angular.z = ...
    (vx/L) * ...
    (tan(steer_front)-tan(steer_rear));


end

== matlab function ATOM_simple_planning_simulator/parking_velocity_smoother2/MATLAB Function ==
  data: trajectory_in input Bus: TrajectoryDataBus size=1; trajectory_out output Bus: TrajectoryDataBus size=1
function trajectory_out = parkingVelocitySmoother(trajectory_in)
%#codegen
%
% Generate the longitudinal velocity and acceleration reference
% for one forward or reverse parking segment.

% Preserve all fields of the original trajectory bus.
trajectory_out = trajectory_in;

% The parking trajectory contains exactly 100 points.
N = 100;

%% 1. Velocity-profile parameters

% v_max       = 0.30; %0.50;   % previously 1.00  % desired maximum parking speed [m/s]
% a_accel_max = 0.25; %0.5;   % previously 1.00   % from velocity_smoother.max_acc

v_max           = 0.80;
v_curve         = 0.30;
steer_threshold = 0.10;

a_accel_max = 0.25;
a_decel_max = 0.50;

% Existing lateral-acceleration limit from velocity_smoother_params.m.
a_lat_max = 1.00;     % maximum lateral acceleration [m/s^2]

% Existing curvature-calculation distance from
% velocity_smoother_params.m.
curvature_calculation_distance = 2.00;   % [m]

%% 2. Read the trajectory data

px = trajectory_in.pose.position.x;
py = trajectory_in.pose.position.y;

% rear_angle = trajectory_in.rear_wheel_angle_rad;

front_angle = trajectory_in.front_wheel_angle_rad;
rear_angle  = trajectory_in.rear_wheel_angle_rad;


% At this stage, the incoming velocity is used only to determine
% whether the segment is forward or reverse.
raw_velocity = trajectory_in.longitudinal_velocity_mps;

%% 3. Determine the segment direction

% Default to forward if no nonzero direction can be found.
gear = 1.0;

for k = 1:N
    if abs(raw_velocity(k)) > 1e-6
        gear = sign(raw_velocity(k));
        break;
    end
end

%% 4. Calculate distance between consecutive trajectory points

ds = zeros(N-1,1);
path_length = 0.0;

for k = 1:N-1
    dx = px(k+1) - px(k);
    dy = py(k+1) - py(k);

    ds(k) = hypot(dx,dy);
    path_length = path_length + ds(k);
end

% Use higher speed only when the active segment is long enough.
% long_segment_threshold = 2.0;   % [m]

% if path_length > long_segment_threshold
%     v_max       = 0.80;   % [m/s]
%     a_accel_max = 0.50;   % [m/s^2]
% end

%% 5. Calculate trajectory curvature

% pathToTrajectory resamples the segment at approximately equal
% distances, so an index separation can represent the requested
% curvature-calculation distance.

point_interval = path_length / (N-1);

idx_dist = 1;

if point_interval > 1e-6
    idx_dist = floor( ...
        curvature_calculation_distance / point_interval);
end

% Three curvature points must remain inside the trajectory.
max_idx_dist = floor((N-1)/2);

idx_dist = max(1,min(idx_dist,max_idx_dist));

curvature = zeros(N,1);

for k = 2:N-1

    idx_prev = k - min(idx_dist,k-1);
    idx_next = k + min(idx_dist,N-k);

    x1 = px(idx_prev);
    y1 = py(idx_prev);

    x2 = px(k);
    y2 = py(k);

    x3 = px(idx_next);
    y3 = py(idx_next);

    d12 = hypot(x2-x1,y2-y1);
    d23 = hypot(x3-x2,y3-y2);
    d31 = hypot(x1-x3,y1-y3);

    denominator = d12*d23*d31;

    if abs(denominator) > 1e-10

        curvature(k) = 2.0 * ( ...
            (x2-x1)*(y3-y1) - ...
            (y2-y1)*(x3-x1)) / denominator;

    else

        % Degenerate or repeated trajectory points.
        curvature(k) = 0.0;

    end
end

% Complete the two boundary values.
curvature(1) = curvature(2);
curvature(N) = curvature(N-1);

%% 6. Build the speed ceiling

% Begin with the requested maximum parking speed.
speed_limit = v_max * ones(N,1);

% Slow down whenever the planned wheels are steering.
for k = 1:N

    steering_activity = max( ...
        abs(front_angle(k)), ...
        abs(rear_angle(k)));

    if steering_activity > steer_threshold
        speed_limit(k) = min(speed_limit(k),v_curve);
    end
end


% Reduce the speed wherever the trajectory curvature would cause the
% lateral acceleration to exceed a_lat_max.
%
% Current 4WS model relation:
%
%     a_lat = vx^2 * curvature / cos(delta_r)
%
% Therefore:
%
%     vx_max = sqrt(a_lat_max*cos(delta_r)/abs(curvature))

for k = 1:N

    kappa = abs(curvature(k));

    if kappa > 1e-6

        cos_rear = cos(rear_angle(k));

        % Numerical protection. With the present steering limits,
        % cos(rear_angle) should remain positive.
        if cos_rear < 1e-6
            cos_rear = 1e-6;
        end

        v_lateral_max = sqrt( ...
            a_lat_max*cos_rear/kappa);

        % The final local ceiling is the smaller of:
        %   1. the 2 m/s parking limit;
        %   2. the curvature-based lateral limit.
        speed_limit(k) = min( ...
            speed_limit(k), ...
            v_lateral_max);
    end
end

%% 7. Backward pass: ensure that the vehicle can stop

speed_backward = speed_limit;

% Every parking segment ends at rest.
speed_backward(N) = 0.0;

for k = N-1:-1:1

    % Maximum speed at point k from which the vehicle can still
    % brake to speed_backward(k+1).
    reachable_speed = sqrt( ...
        speed_backward(k+1)^2 + ...
        2.0*a_decel_max*ds(k));

    speed_backward(k) = min( ...
        speed_backward(k), ...
        reachable_speed);
end

%% 8. Forward pass: enforce the acceleration limit

speed_magnitude = speed_backward;

% Every segment starts at rest, including after a gear reversal.
speed_magnitude(1) = 0.0;

for k = 2:N

    % Maximum speed reachable from the previous point without
    % exceeding a_accel_max.
    reachable_speed = sqrt( ...
        speed_magnitude(k-1)^2 + ...
        2.0*a_accel_max*ds(k-1));

    speed_magnitude(k) = min( ...
        speed_backward(k), ...
        reachable_speed);
end

%% 9. Calculate the compatible acceleration reference

acceleration_magnitude = zeros(N,1);

for k = 1:N-1

    if ds(k) > 1e-6

        acceleration_magnitude(k) = ...
            (speed_magnitude(k+1)^2 - ...
             speed_magnitude(k)^2) / ...
            (2.0*ds(k));

    else

        % Protect against duplicate consecutive points.
        acceleration_magnitude(k) = 0.0;

    end
end

% The vehicle remains stopped at the segment endpoint.
acceleration_magnitude(N) = 0.0;

%% 10. Apply the forward or reverse sign

trajectory_out.longitudinal_velocity_mps = ...
    gear*speed_magnitude;

trajectory_out.acceleration_mps2 = ...
    gear*acceleration_magnitude;

end

== matlab function ATOM_simple_planning_simulator/steeringRatetoAngle2/steeringRateToAngle ==
  settings: updateMethod=DISCRETE  sampleTime=0.04
  data: df_rate_cmd input; df_angle_cmd output; dr_rate_cmd input; df_measured input; dr_measured input; sample_time input; steer_rate_limit input; steer_angle_limit input; dr_angle_cmd output
function [df_angle_cmd, dr_angle_cmd] = steeringRateToAngle( ...
    df_rate_cmd, dr_rate_cmd, df_measured, dr_measured, ...
    sample_time, steer_rate_limit, steer_angle_limit)

persistent df_command_state dr_command_state

% Initialize the commanded angles from the measured wheel angles.
if isempty(df_command_state)
    df_command_state = max( ...
        -steer_angle_limit, ...
        min(steer_angle_limit,df_measured));

    dr_command_state = max( ...
        -steer_angle_limit, ...
        min(steer_angle_limit,dr_measured));
end

% Apply hard steering-rate limits.
front_rate = max( ...
    -steer_rate_limit, ...
    min(steer_rate_limit,df_rate_cmd));

rear_rate = max( ...
    -steer_rate_limit, ...
    min(steer_rate_limit,dr_rate_cmd));

% Integrate rates into desired steering angles.
df_command_state = df_command_state + sample_time*front_rate;
dr_command_state = dr_command_state + sample_time*rear_rate;

% Apply hard steering-angle limits.
df_command_state = max( ...
    -steer_angle_limit, ...
    min(steer_angle_limit,df_command_state));

dr_command_state = max( ...
    -steer_angle_limit, ...
    min(steer_angle_limit,dr_command_state));

df_angle_cmd = df_command_state;
dr_angle_cmd = dr_command_state;

end
